simulink model "cascade_pid_motor"  (R2025b)
settings: Solver=ode45  StartTime=0.0  StopTime=16  MaxStep=0.002  RelTol=1e-6  AbsTol=1e-8
model workspace (MAT data in the model file):
  J = 0.01
  Kd_pos = 0.05
  Ke = 0.1
  Ki_pos = 3
  Ki_speed = 40
  Kp_pos = 4
  Kp_speed = 4
  Kt = 0.1
  L = 0.01
  N_pos = 30
  R = 1
  b = 0.001
  load_torque = 0.05
  speed_limit = 8
  theta_change = -3.14159265359
  theta_step = 1.57079632679
  voltage_limit = 24
libraries: slpidlib x2
settings Model: Creator=alosw  LastModifiedBy=alosw

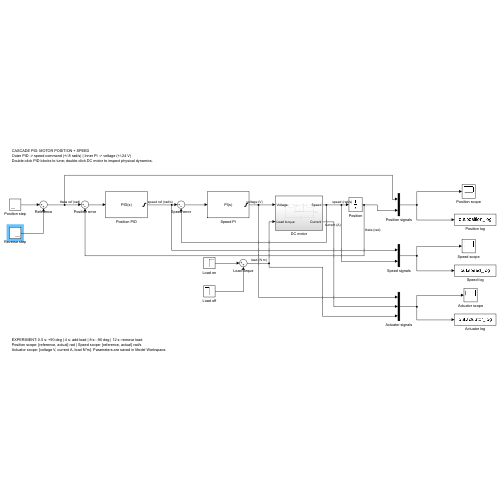
[thumbnail: Simulink's stored preview of the top-level diagram]
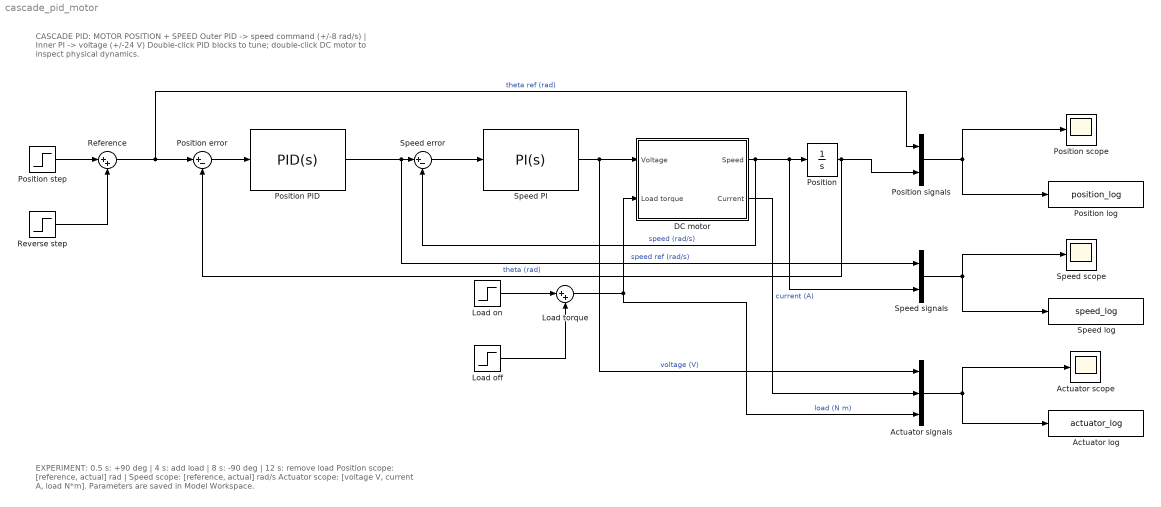
== system cascade_pid_motor ==
  note: CASCADE PID: MOTOR POSITION + SPEED
      | Outer PID -> speed command (+/-8 rad/s) | Inner PI -> voltage (+/-24 V)
      | Double-click PID blocks to tune; double-click DC motor to inspect physical dynamics.
  note: EXPERIMENT: 0.5 s: +90 deg | 4 s: add load | 8 s: -90 deg | 12 s: remove load
      | Position scope: [reference, actual] rad | Speed scope: [reference, actual] rad/s
      | Actuator scope: [voltage V, current A, load N*m]. Parameters are saved in Model Workspace.
  Actuator log : ToWorkspace  VariableName=actuator_log  SaveFormat=Timeseries  SampleTime=-1
  Actuator scope : Scope
  Actuator signals : Mux  Inputs=3
  DC motor : Subsystem
  Load off : Step  Time=12  After=-load_torque  SampleTime=0
  Load on : Step  Time=4  After=load_torque  SampleTime=0
  Load torque : Sum  Inputs=|++
  Position : Integrator
  Position PID : slpidlib/PID Controller  Controller=PID  Form=Parallel  TimeDomain=Continuous-time  UseExternalTs=off  SampleTime=-1  IntegratorMethod=Forward Euler  FilterMethod=Forward Euler  ControllerParametersSource=internal  P=Kp_pos  I=Ki_pos  UseKiTs=off  D=Kd_pos  UseExternalDerivativeSource=off  N=N_pos  UseFilter=on  TunerSelectOption=Transfer Function Based (PID Tuner App)  InitialConditionSource=internal  InitialConditionForIntegrator=0  InitialConditionForFilter=0  DifferentiatorICPrevScaledInput=0  ExternalReset=none  TrackingMode=off  Kt=1  LimitOutput=on  SatLimitsSource=internal  UpperSaturationLimit=speed_limit  LowerSaturationLimit=-speed_limit  LinearizeAsGain=on  AntiWindupMode=back-calculation  Kb=1  LimitIntegrator=off  UpperIntegratorSaturationLimit=inf  LowerIntegratorSaturationLimit=-inf  POutMin=[]  POutMax=[]  IOutMin=[]  IOutMax=[]  DOutMin=[]  DOutMax=[]  NOutMin=[]  NOutMax=[]  SumOutMin=[]  SumOutMax=[]  SaturationOutMin=[]  SaturationOutMax=[]  PParamMin=[]  PParamMax=[]  IParamMin=[]  IParamMax=[]  DParamMin=[]  DParamMax=[]  NParamMin=[]  NParamMax=[]  KbParamMin=[]  KbParamMax=[]  KtParamMin=[]  KtParamMax=[]  KbOutMin=[]  KbOutMax=[]  KtOutMin=[]  KtOutMax=[]  IntegratorOutMin=[]  IntegratorOutMax=[]  FilterOutMin=[]  FilterOutMax=[]  SumI1OutMin=[]  SumI1OutMax=[]  SumI2OutMin=[]  SumI2OutMax=[]  SumI3OutMin=[]  SumI3OutMax=[]  SumI4OutMin=[]  SumI4OutMax=[]  SumDOutMin=[]  SumDOutMax=[]  DifferentiatorOutMin=[]  DifferentiatorOutMax=[]  FilterDiffOutCoefMin=[]  FilterDiffOutCoefMax=[]  ReciprocalOutMin=[]  ReciprocalOutMax=[]  SumDenOutMin=[]  SumDenOutMax=[]  SumNumOutMin=[]  SumNumOutMax=[]  DivideOutMin=[]  DivideOutMax=[]  UdiffTsProdOutMin=[]  UdiffTsProdOutMax=[]  NTsProdOutMin=[]  NTsProdOutMax=[]  UintegralTsProdOutMin=[]  UintegralTsProdOutMax=[]  UngainTsProdOutMin=[]  UngainTsProdOutMax=[]  ClampingZeroOutDataTypeStr=Inherit: Inherit via back propagation  ClampingZeroOutMin=[]  ClampingZeroOutMax=[]  FilterDenConstantOutDataTypeStr=Inherit: Inherit via back propagation  FilterDenConstantOutMin=[]  FilterDenConstantOutMax=[]  PCopyOutDataTypeStr=Inherit: Inherit via back propagation  PCopyOutMin=[]  PCopyOutMax=[]  NCopyOutDataTypeStr=Inherit: Inherit via back propagation  NCopyOutMin=[]  NCopyOutMax=[]  IntegratorContinuousStateAttributes=''  IntegratorStateMustResolveToSignalObject=off  IntegratorRTWStateStorageClass=Auto  FilterContinuousStateAttributes=''  FilterStateMustResolveToSignalObject=off  FilterRTWStateStorageClass=Auto  ParallelPVariant=InternalParameters  IdealPVariant=Disabled  IVariant=InternalParameters  DVariant=InternalParameters  IntegratorVariant=Continuous  SatVariant=Enabled  AWVariant=BackCalculation  PCopyVariant=Disabled  TRVariant=Disabled  FdbkBlocksVariant=Forward  IdealPFdbkVariant=Disabled  SatFdbkVariant=Disabled  DerivativeFilterVariant=ContFilter  NVariant=InternalParameters  NCopyVariant=Disabled  FilterICVariant=InternalICsFilter  IntegratorICVariant=InternalICs  ExternalResetVariant=Disabled  TRSumVariant=Passthrough  SumFdbkVariant=Disabled  SumVariant=Sum_PID  TsampFilterVariant=InternalTs  TsampNgainVariant=Passthrough  TsampIntegralVariant=Disabled_SignalSpec  ExternalSaturationOutDataTypeStr=Inherit: Same as second input  DerivativeSourceVariant=ErrorSignal  PreIntVariant=InternalPreInt
  Position error : Sum  Inputs=|+-
  Position log : ToWorkspace  VariableName=position_log  SaveFormat=Timeseries  SampleTime=-1
  Position scope : Scope
      settings: ActiveDisplayYMinimum=-2.3475131315570232  ActiveDisplayYMaximum=2.2002192522469528
  Position signals : Mux  Inputs=2
  Position step : Step  Time=0.5  After=theta_step  SampleTime=0
  Reference : Sum  Inputs=|++
  Reverse step : Step  Time=8  After=theta_change  SampleTime=0
  Speed PI : slpidlib/PID Controller  Controller=PI  Form=Parallel  TimeDomain=Continuous-time  UseExternalTs=off  SampleTime=-1  IntegratorMethod=Forward Euler  FilterMethod=Forward Euler  ControllerParametersSource=internal  P=Kp_speed  I=Ki_speed  UseKiTs=off  D=0  UseExternalDerivativeSource=off  N=100  UseFilter=on  TunerSelectOption=Transfer Function Based (PID Tuner App)  InitialConditionSource=internal  InitialConditionForIntegrator=0  InitialConditionForFilter=0  DifferentiatorICPrevScaledInput=0  ExternalReset=none  TrackingMode=off  Kt=1  LimitOutput=on  SatLimitsSource=internal  UpperSaturationLimit=voltage_limit  LowerSaturationLimit=-voltage_limit  LinearizeAsGain=on  AntiWindupMode=back-calculation  Kb=20  LimitIntegrator=off  UpperIntegratorSaturationLimit=inf  LowerIntegratorSaturationLimit=-inf  POutMin=[]  POutMax=[]  IOutMin=[]  IOutMax=[]  DOutMin=[]  DOutMax=[]  NOutMin=[]  NOutMax=[]  SumOutMin=[]  SumOutMax=[]  SaturationOutMin=[]  SaturationOutMax=[]  PParamMin=[]  PParamMax=[]  IParamMin=[]  IParamMax=[]  DParamMin=[]  DParamMax=[]  NParamMin=[]  NParamMax=[]  KbParamMin=[]  KbParamMax=[]  KtParamMin=[]  KtParamMax=[]  KbOutMin=[]  KbOutMax=[]  KtOutMin=[]  KtOutMax=[]  IntegratorOutMin=[]  IntegratorOutMax=[]  FilterOutMin=[]  FilterOutMax=[]  SumI1OutMin=[]  SumI1OutMax=[]  SumI2OutMin=[]  SumI2OutMax=[]  SumI3OutMin=[]  SumI3OutMax=[]  SumI4OutMin=[]  SumI4OutMax=[]  SumDOutMin=[]  SumDOutMax=[]  DifferentiatorOutMin=[]  DifferentiatorOutMax=[]  FilterDiffOutCoefMin=[]  FilterDiffOutCoefMax=[]  ReciprocalOutMin=[]  ReciprocalOutMax=[]  SumDenOutMin=[]  SumDenOutMax=[]  SumNumOutMin=[]  SumNumOutMax=[]  DivideOutMin=[]  DivideOutMax=[]  UdiffTsProdOutMin=[]  UdiffTsProdOutMax=[]  NTsProdOutMin=[]  NTsProdOutMax=[]  UintegralTsProdOutMin=[]  UintegralTsProdOutMax=[]  UngainTsProdOutMin=[]  UngainTsProdOutMax=[]  ClampingZeroOutDataTypeStr=Inherit: Inherit via back propagation  ClampingZeroOutMin=[]  ClampingZeroOutMax=[]  FilterDenConstantOutDataTypeStr=Inherit: Inherit via back propagation  FilterDenConstantOutMin=[]  FilterDenConstantOutMax=[]  PCopyOutDataTypeStr=Inherit: Inherit via back propagation  PCopyOutMin=[]  PCopyOutMax=[]  NCopyOutDataTypeStr=Inherit: Inherit via back propagation  NCopyOutMin=[]  NCopyOutMax=[]  IntegratorContinuousStateAttributes=''  IntegratorStateMustResolveToSignalObject=off  IntegratorRTWStateStorageClass=Auto  FilterContinuousStateAttributes=''  FilterStateMustResolveToSignalObject=off  FilterRTWStateStorageClass=Auto  ParallelPVariant=InternalParameters  IdealPVariant=Disabled  IVariant=InternalParameters  DVariant=Disabled  IntegratorVariant=Continuous  SatVariant=Enabled  AWVariant=BackCalculation  PCopyVariant=Disabled  TRVariant=Disabled  FdbkBlocksVariant=Forward  IdealPFdbkVariant=Disabled  SatFdbkVariant=Disabled  DerivativeFilterVariant=Disabled  NVariant=Disabled  NCopyVariant=Disabled_SignalSpec  FilterICVariant=Disabled  IntegratorICVariant=InternalICs  ExternalResetVariant=Disabled  TRSumVariant=Passthrough  SumFdbkVariant=Disabled  SumVariant=Sum_PI  TsampFilterVariant=InternalTs  TsampNgainVariant=Passthrough  TsampIntegralVariant=Disabled_SignalSpec  ExternalSaturationOutDataTypeStr=Inherit: Same as second input  DerivativeSourceVariant=Disabled  PreIntVariant=InternalPreInt
  Speed error : Sum  Inputs=|+-
  Speed log : ToWorkspace  VariableName=speed_log  SaveFormat=Timeseries  SampleTime=-1
  Speed scope : Scope
      settings: ActiveDisplayYMinimum=-14.994120314241314  ActiveDisplayYMaximum=1.2083845497026529
  Speed signals : Mux  Inputs=2
  wires:
  Position signals/1 -> Position scope/1, Position log/1
  Speed signals/1 -> Speed scope/1, Speed log/1
  Actuator signals/1 -> Actuator scope/1, Actuator log/1
  Position step/1 -> Reference/1
  Reverse step/1 -> Reference/2
  Reference/1 -> Position error/1, Position signals/1  "theta ref (rad)"
  Position error/1 -> Position PID/1
  Position PID/1 -> Speed signals/1, Speed error/1  "speed ref (rad/s)"
  Speed error/1 -> Speed PI/1
  Speed PI/1 -> Actuator signals/1, DC motor/1(Voltage)  "voltage (V)"
  Load on/1 -> Load torque/1
  Load off/1 -> Load torque/2
  Load torque/1 -> Actuator signals/3, DC motor/2(Load torque)  "load (N m)"
  DC motor/1(Speed) -> Position/1, Speed signals/2, Speed error/2  "speed (rad/s)"
  Position/1 -> Position signals/2, Position error/2  "theta (rad)"
  DC motor/2(Current) -> Actuator signals/2  "current (A)"

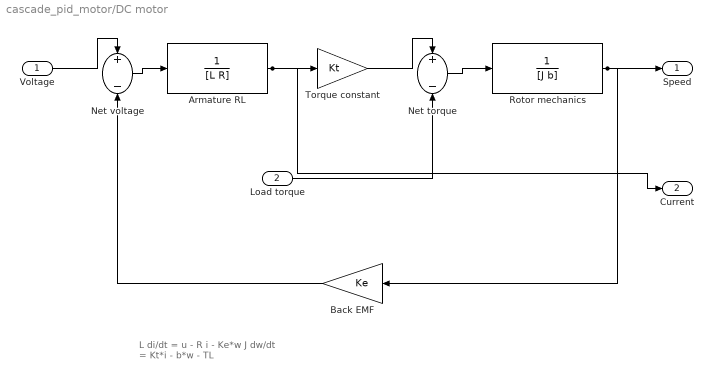
== system cascade_pid_motor/DC motor ==
  note: L di/dt = u - R i - Ke*w
      | J dw/dt = Kt*i - b*w - TL
  Voltage : Inport
  Load torque : Inport  Port=2
  Armature RL : TransferFcn  Numerator=1  Denominator=[L R]
  Back EMF : Gain  Gain=Ke
  Net torque : Sum  Inputs=+-
  Net voltage : Sum  Inputs=+-
  Rotor mechanics : TransferFcn  Numerator=1  Denominator=[J b]
  Torque constant : Gain  Gain=Kt
  Speed : Outport
  Current : Outport  Port=2
  wires:
  Voltage/1 -> Net voltage/1
  Net voltage/1 -> Armature RL/1
  Armature RL/1 -> Torque constant/1, Current/1
  Torque constant/1 -> Net torque/1
  Load torque/1 -> Net torque/2
  Net torque/1 -> Rotor mechanics/1
  Rotor mechanics/1 -> Speed/1, Back EMF/1
  Back EMF/1 -> Net voltage/2
